simulink model "plant"  (R2026a)
settings: Solver=ode4  StopTime=2  FixedStep=0.001
undefined symbols (not defined in the file): P
settings Model: Creator=muthi  LastModifiedBy=muthi

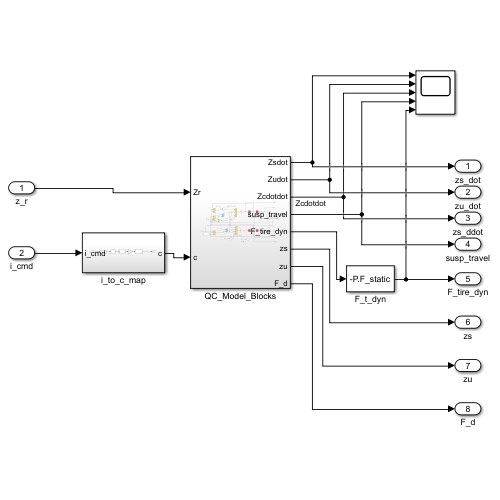
[thumbnail: Simulink's stored preview of the top-level diagram]
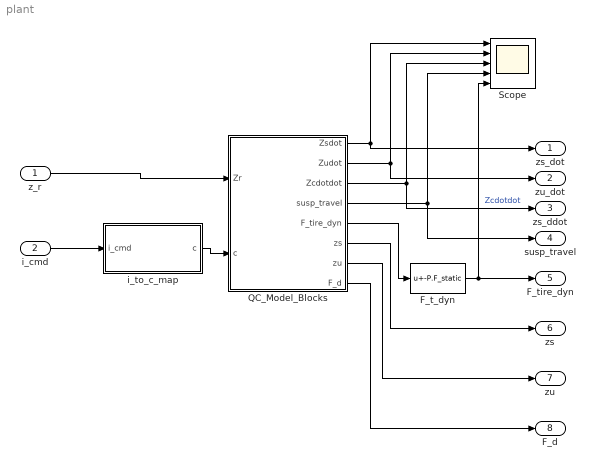
== system plant ==
  z_r : Inport
  i_cmd : Inport  Port=2
  F_t_dyn : Bias  Bias=-P.F_static  SaturateOnIntegerOverflow=off
  QC_Model_Blocks : Subsystem
  Scope : Scope  NumInputPorts=5
      settings: ActiveDisplayYMinimum=-5.1160117044528832E-13  ActiveDisplayYMaximum=5.69370251429538E-14
  i_to_c_map : Subsystem
  zs_dot : Outport
  zu_dot : Outport  Port=2
  zs_ddot : Outport  Port=3
  susp_travel : Outport  Port=4
  F_tire_dyn : Outport  Port=5
  zs : Outport  Port=6
  zu : Outport  Port=7
  F_d : Outport  Port=8
  wires:
  QC_Model_Blocks/3(Zcdotdot) -> zs_ddot/1, Scope/3  "Zcdotdot"
  QC_Model_Blocks/4(susp_travel) -> susp_travel/1, Scope/4
  QC_Model_Blocks/1(Zsdot) -> zs_dot/1, Scope/1
  QC_Model_Blocks/2(Zudot) -> zu_dot/1, Scope/2
  QC_Model_Blocks/5(F_tire_dyn) -> F_t_dyn/1
  F_t_dyn/1 -> Scope/5, F_tire_dyn/1
  z_r/1 -> QC_Model_Blocks/1(Zr)
  i_cmd/1 -> i_to_c_map/1(i_cmd)
  i_to_c_map/1(c) -> QC_Model_Blocks/2(c)
  QC_Model_Blocks/8(F_d) -> F_d/1
  QC_Model_Blocks/7(zu) -> zu/1
  QC_Model_Blocks/6(zs) -> zs/1

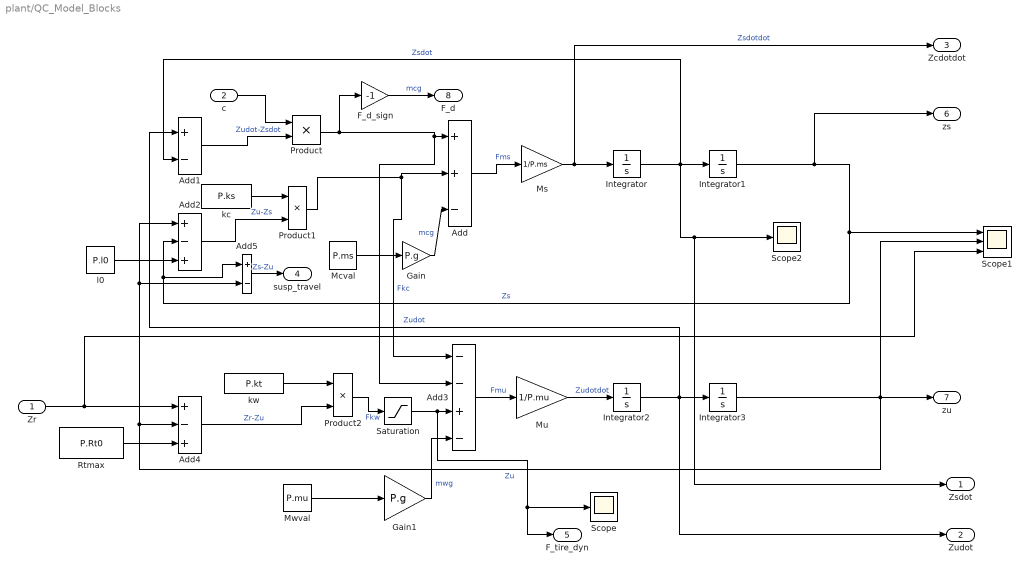
== system plant/QC_Model_Blocks ==
  Zr : Inport
  c : Inport  Port=2
  Add : Sum  Inputs=++-
  Add1 : Sum  Inputs=+-
  Add2 : Sum  Inputs=+-+
  Add3 : Sum  Inputs=--+-
  Add4 : Sum  Inputs=+-+
  Add5 : Sum  Inputs=+-
  F_d_sign : Gain  Gain=-1
  Gain : Gain  Gain=P.g
  Gain1 : Gain  Gain=P.g
  Integrator{,1..3} (4 alike) : Integrator
  Mcval : Constant  Value=P.ms
  Ms : Gain  Gain=1/P.ms
  Mu : Gain  Gain=1/P.mu
  Mwval : Constant  Value=P.mu
  Product : Product
  Product1 : Product
  Product2 : Product
  Rtmax : Constant  Value=P.Rt0
  Saturation : Saturate  UpperLimit=inf  LowerLimit=0
  Scope : Scope
      settings: ActiveDisplayYMinimum=2594.745  ActiveDisplayYMaximum=2594.7450000000003  DataLoggingVariableName=ScopeData3
  Scope1 : Scope  NumInputPorts=3
      settings: ActiveDisplayYMinimum=-0.099617790090906155  ActiveDisplayYMaximum=0.19555431394271514
  Scope2 : Scope
      settings: ActiveDisplayYMinimum=-1.0710287209694067  ActiveDisplayYMaximum=0.54545782927297148  DataLoggingVariableName=ScopeData6
  kc : Constant  Value=P.ks
  kw : Constant  Value=P.kt
  l0 : Constant  Value=P.l0
  Zsdot : Outport
  Zudot : Outport  Port=2
  Zcdotdot : Outport  Port=3
  susp_travel : Outport  Port=4
  F_tire_dyn : Outport  Port=5
  zs : Outport  Port=6
  zu : Outport  Port=7
  F_d : Outport  Port=8
  wires:
  Ms/1 -> Zcdotdot/1, Integrator/1  "Zsdotdot"
  Mwval/1 -> Gain1/1
  Add3/1 -> Mu/1  "Fmu"
  Mcval/1 -> Gain/1
  Integrator1/1 -> zs/1, Scope1/1, Add2/2, Add5/1  "Zs"
  Add/1 -> Ms/1  "Fms"
  Product1/1 -> Add3/1, Add/2  "Fkc"
  kw/1 -> Product2/1
  Integrator3/1 -> zu/1, Scope1/2, Add5/2, Add2/1, Add4/2  "Zu"
  Integrator/1 -> Zsdot/1, Scope2/1, Add1/2, Integrator1/1  "Zsdot"
  Integrator2/1 -> Zudot/1, Add1/1, Integrator3/1  "Zudot"
  Add4/1 -> Product2/2  "Zr-Zu"
  Mu/1 -> Integrator2/1  "Zudotdot"
  Zr/1 -> Scope1/3, Add4/1
  Add2/1 -> Product1/2  "Zu-Zs"
  Gain/1 -> Add/3  "mcg"
  Rtmax/1 -> Add4/3
  Product2/1 -> Saturation/1  "Fkw"
  Gain1/1 -> Add3/4  "mwg"
  kc/1 -> Product1/1
  Saturation/1 -> F_tire_dyn/1, Scope/1, Add3/3
  Product/1 -> F_d_sign/1, Add3/2, Add/1
  Add1/1 -> Product/2  "Zudot-Zsdot"
  c/1 -> Product/1
  l0/1 -> Add2/3
  Add5/1 -> susp_travel/1  "Zs-Zu"
  F_d_sign/1 -> F_d/1  "mcg"

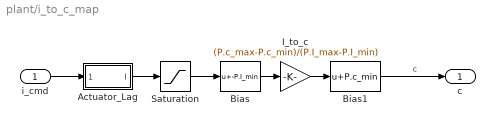
== system plant/i_to_c_map ==
  i_cmd : Inport
  Actuator_Lag : Subsystem
  Bias : Bias  Bias=-P.I_min  SaturateOnIntegerOverflow=off
  Bias1 : Bias  Bias=P.c_min  SaturateOnIntegerOverflow=off
  I_to_c : Gain  Gain=(P.c_max-P.c_min)/(P.I_max-P.I_min)
  Saturation : Saturate  UpperLimit=P.I_max  LowerLimit=P.I_min
  c : Outport
  wires:
  Bias/1 -> I_to_c/1
  Bias1/1 -> c/1  "c"
  I_to_c/1 -> Bias1/1
  Saturation/1 -> Bias/1
  Actuator_Lag/1(I) -> Saturation/1
  i_cmd/1 -> Actuator_Lag/1(i_cmd)

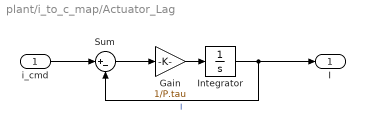
== system plant/i_to_c_map/Actuator_Lag ==
  i_cmd : Inport
  Gain : Gain  Gain=1/P.tau
  Integrator : Integrator  InitialCondition=P.I_default
  Sum : Sum  Inputs=|+-
  I : Outport
  wires:
  Integrator/1 -> I/1, Sum/2  "I"
  Gain/1 -> Integrator/1
  i_cmd/1 -> Sum/1
  Sum/1 -> Gain/1
